simulink model "CHB_inverter_PEE_PROJECT"  (R2026a)
settings: Solver=VariableStepAuto  StopTime=0.04
libraries: nesl_utility x15, ee_lib x10, fl_lib x8, simulink x4
settings Model: Creator=THIRUPUGAZHL S D  LastModifiedBy=THIRUPUGAZHL S D

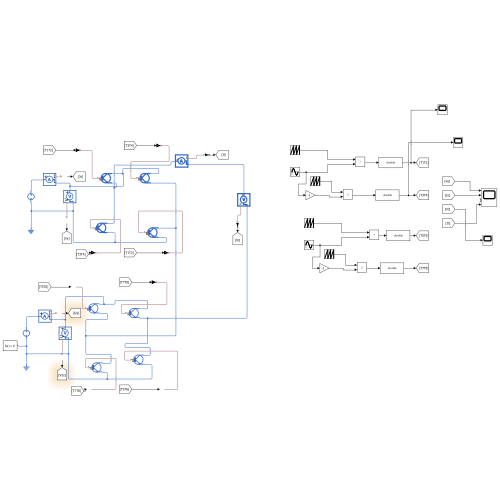
[thumbnail: Simulink's stored preview of the top-level diagram]
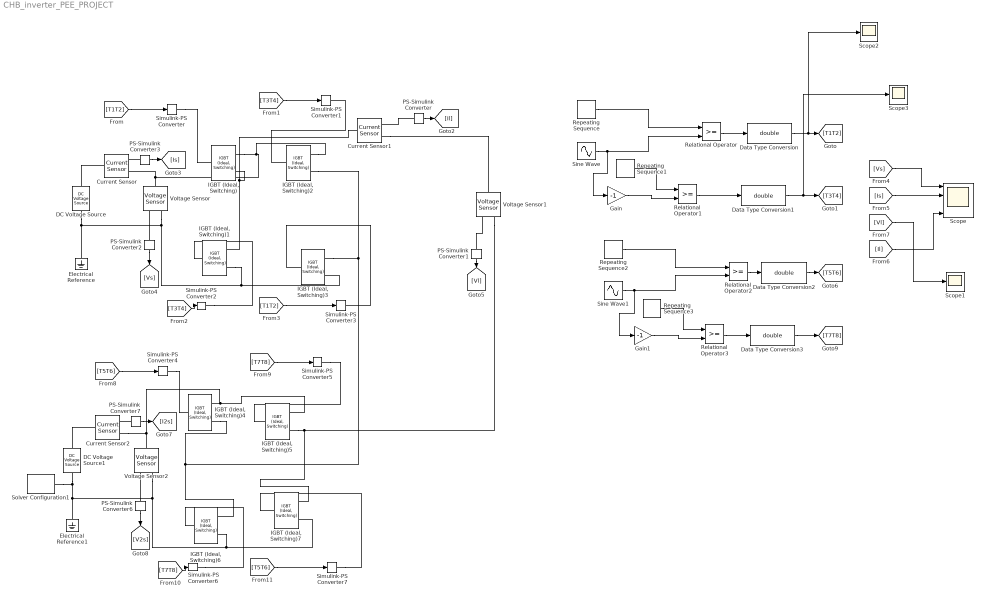
== system CHB_inverter_PEE_PROJECT ==
  Current Sensor : fl_lib/Electrical/Electrical Sensors/Current Sensor
  Current Sensor1 : fl_lib/Electrical/Electrical Sensors/Current Sensor
  Current Sensor2 : fl_lib/Electrical/Electrical Sensors/Current Sensor
  DC Voltage Source : ee_lib/Additional Components/SPICE Sources/DC Voltage Source  DC=50 V
  DC Voltage Source1 : ee_lib/Additional Components/SPICE Sources/DC Voltage Source  DC=50 V
  Data Type Conversion{,1..3} (4 alike) : DataTypeConversion  OutDataTypeStr=double  SaturateOnIntegerOverflow=off  RndMeth=Floor
  Electrical Reference : fl_lib/Electrical/Electrical Elements/Electrical Reference
  Electrical Reference1 : fl_lib/Electrical/Electrical Elements/Electrical Reference
  Gain : Gain  Gain=-1
  Gain1 : Gain  Gain=-1
  IGBT (Ideal, Switching){,1..7} (8 alike) : ee_lib/Semiconductors & Converters/IGBT (Ideal, Switching)  port_option=ee.enum.controlport.ps  Vf=0.8 V  Ron=0.001 Ohm  Goff=1e-5 1/Ohm  Vth=0.5 V  diode_param=ee.enum.semiconductors.protectionDiode.external  diode_Vf=0.8 V  diode_Ron=0.001 Ohm  diode_Goff=1e-5 1/Ohm  diode_C=50e-9 F  diode_iRM=-235 A  diode_iF=300 A  diode_idot=-50 A/us  diode_trr_param=ee.enum.converters.diodeReverseParam.trr_factor  diode_trr_factor=3  diode_trr=15 us  diode_Qrr=1500 s*uA  ice_specify=off  ice_priority=None  ice=0 A  ice_nominal_specify=off  ice_nominal_value=1  ice_nominal_unit=A  vce_specify=off  vce_priority=None  vce=0 V  vce_nominal_specify=off  vce_nominal_value=1  vce_nominal_unit=V  vge_specify=off  vge_priority=None  vge=0 V  vge_nominal_specify=off  vge_nominal_value=1  vge_nominal_unit=V  thermal_loss_option=ee.enum.converters.thermalLossOption.constantvalues  Von_data=[0, .1, .6, .8, 1, 1.3, 1.6, 2, 2.4; 0, .1, .7, 1, 1.2, 1.5, 1.9, 2.4, 2.8] V  Tj=[298.15, 398.15] K  Iout_data=[0, .1, 1, 5, 10, 20, 40, 70, 100] A  tabulateWithVce=false  Eon_data=[0, .0024, .024, .12, .2, .48, 1.04, 2.16, 3.24; 0, .003, .03, .15, .25, .6, 1.3, 2.7, 4.05] * 1e-3 J  Eoff_data=[0, .0007, .0066, .033, .066, .17, .33, .83, 1.5; 0, .001, .01, .05, .1, .25, .5, 1.2, 2.2] * 1e-3 J  Eon_data_3D=[zeros(2, 9, 3)] J  Eoff_data_3D=[zeros(2, 9, 3)] J  Tj_loss=[298.15, 398.15] K  Iout_data_loss=[0, .1, 1, 5, 10, 20, 40, 70, 100] A  Vce_loss=[0, 150, 300] V  Eon_scalar=22.86e-3 J  Eoff_scalar=17.14e-3 J  Voff=300 V  Iout_scalar=600 A  useCurrentFromPreviousCycle=false  useVoltageFromPreviousCycle=false  diodeModelType=ee.enum.converters.diodeModelType.pwl  diodeTableType=ee.enum.diode.tableType.IfMat  diode_ReverseIVType=ee.enum.diode.diodeReverseIV.constant  diode_IfMat=[.07, .12, .19, 1.75, 4.24, 7.32, 11.2; .16, .3, .72, 2.14, 4.02, 6.35, 9.12] A  diode_VfMat=[.9, 1.15, 1.25, 1.5, 1.75, 2.17, 2.6, 2.85; .58, .68, .75, 1.1, 1.38, 1.77, 2.27, 2.7] V  diode_TjVec=[25, 125] degC  diode_VfVec=[.5, .7, .9, 1.3, 1.7, 2.1, 2.5] V  diode_IfVec=[.1, .2, .5, 1, 2, 4, 7, 10] A  diode_IrMat=[1e-06, 2e-06, 5e-06, 1e-05, 2.5e-05, 5e-05, .0001; 2e-06, 5e-06, 1e-05, 4e-05, 8e-05, .0002, .0005] A  diode_VrMat=[10, 100, 200, 250, 300, 325, 350; 10, 70, 160, 220, 270, 300, 320] V  diode_VrVec=[10, 20, 40, 50, 70, 80, 100] V  diode_IrVec=[1e-06, 2e-06, 5e-06, 1e-05, 2e-05, 5e-05, .0001] A  diode_Vr=-600 V  diode_Ls=150 nH  diode_Erec=0.03 J  diode_rec_loss_model=ee.enum.diode.reverseRecoveryModelTabulateUpTo3D.fixed  diode_ErecVal=0 J  diode_scaleWithIandV=true  diode_ErecMat=zeros(2, 3) J  diodeErecMat3D=zeros(2, 3, 2) J  diode_TjrecVec=[298.15, 398.15] K  diode_IfrecVec=[.1, 1, 10] A  diodeVrecVec=[0, 100] V  diode_IrecVal=10 A  diode_VrecVal=10 V  diode_tFilter=1 / 1000 / 100 s  separateThermalPortForDiode=false  thermal_network_parameterization=ee.enum.thermalNetworkTopology.external  Rth=[.08, .5] K/W  Rth_Cauer=[.08, .1, .5] K/W  Rth_Foster=[.08, .14, .22, .16] K/W  thermal_mass_parameterization=ee.enum.thermalNetwork.timeconstant  thermal_mass=[.01, .5] J/K  thermal_mass_Cauer=[.01, .1, .5] J/K  thermal_mass_Foster=[.001, .005, .05, .5] J/K  thermal_time_constant=[.001, .2] s  thermal_time_constant_Cauer=[.001, .1, .2] s  thermal_time_constant_Foster=[7e-05, .0007, .01, .08] s  thermal_mass_initial_temperatures=[25, 25] degC  thermal_mass_initial_temperatures_Cauer=[25, 25, 25] degC  junction_thermal_mass=0.01 J/K  Tvec_initial_Foster=[25, 25, 25, 25] degC  RthDiode=[.03, .2] K/W  RthCauerDiode=[.03, .1, .2] K/W  RthFosterDiode=[.03, .2] K/W  thermalMassDiode=[3, 25] J/K  thermalMassCauerDiode=[3, 10, 25] J/K  thermalMassFosterDiode=[33, 50] J/K  thermalTauDiode=[.1, 5] s  thermalTauCauerDiode=[.1, 1, 5] s  thermalTauFosterDiode=[1, 10] s  thermalMassInitTempDiode=[25, 25] degC  thermalMassInitTempCauerDiode=[25, 25, 25] degC  junctionthermalMassDiode=0.1 J/K  TVecInitialFosterDiode=[25, 25, 25, 25] degC  no_thermal_network=ee.enum.enable.no  IGBT_junction_temperature_specify=off  IGBT_junction_temperature_priority=None  IGBT_junction_temperature=25 degC  IGBT_junction_temperature_nominal_specify=off  IGBT_junction_temperature_nominal_value=1  IGBT_junction_temperature_nominal_unit=degC  diode_junction_temperature_specify=off  diode_junction_temperature_priority=None  diode_junction_temperature=25 degC  diode_junction_temperature_nominal_specify=off  diode_junction_temperature_nominal_value=1  diode_junction_temperature_nominal_unit=degC  Qj_specify=off  Qj_priority=None  Qj=0 W  Qj_nominal_specify=off  Qj_nominal_value=1  Qj_nominal_unit=W  accumulatedSwitchingLosses_specify=off  accumulatedSwitchingLosses_priority=None  accumulatedSwitchingLosses=0 J
  PS-Simulink Converter{,1..3,6..7} (6 alike) : nesl_utility/PS-Simulink Converter  PhysicalDomain=network_engine_domain  SubClassName=ps_output  LeftPortType=input  RightPortType=output  PseudoPeriodic=off  Frequencies=[]  VectorFormat=inherit  Unit=inherit  AffineConversion=off
  Relational Operator{,1..3} (4 alike) : RelationalOperator  OutDataTypeStr=boolean  RndMeth=Simplest  InputSameDT=off
  Repeating Sequence : simulink/Sources/Repeating Sequence  rep_seq_t=[0 1]  rep_seq_y=[0 1]
  Repeating Sequence1 : simulink/Sources/Repeating Sequence  rep_seq_t=[0 1]  rep_seq_y=[0 1]
  Repeating Sequence2 : simulink/Sources/Repeating Sequence  rep_seq_t=[0 1]  rep_seq_y=[1 2]
  Repeating Sequence3 : simulink/Sources/Repeating Sequence  rep_seq_t=[0 1]  rep_seq_y=[1 2]
  Scope : Scope  NumInputPorts=4
      settings: ActiveDisplayYMinimum=40  ActiveDisplayYMaximum=60
  Scope1 : Scope
      settings: ActiveDisplayYMinimum=-60.499998790000006  ActiveDisplayYMaximum=60.499998790000006
  Scope2 : Scope
      settings: ActiveDisplayYMinimum=-1  ActiveDisplayYMaximum=1  DataLoggingVariableName=ScopeData2
  Scope3 : Scope
      settings: ActiveDisplayYMinimum=-0.12499999999999997  ActiveDisplayYMaximum=1.125  DataLoggingVariableName=ScopeData3
  Simulink-PS Converter{,1..7} (8 alike) : nesl_utility/Simulink-PS Converter  PhysicalDomain=network_engine_domain  SubClassName=ps_input  LeftPortType=input  RightPortType=output  PseudoPeriodic=off  Frequencies=[]  NoiseDistribution=none  NoiseParameters=[]  Unit=1  AffineConversion=off  FilteringAndDerivatives=provide  SimscapeFilterOrder=1  InputFilterTimeConstant=0.001  UdotUserProvided=0
  Sine Wave : Sin  Amplitude=2  Frequency=314  SampleTime=0
  Sine Wave1 : Sin  Amplitude=2  Frequency=314  SampleTime=0
  Solver Configuration1 : nesl_utility/Solver Configuration  PhysicalDomain=network_engine_domain  SubClassName=solver  LeftPortType=input  RightPortType=generic  Tones=[]  Harmonics=[]  SimulateNoise=off  Profile=off  UseLocalSampling=off  EnableSwitchedLinearOptims=on  FrequencyDomain=off  UseCCode=off  RelTol=0.001  AbsTol=0.001  MinStep=1e-09  ToWorkspace=off  RevertToSquareIcSolve=off  NumHomotopyIterations=100  PhasorMode=off  PhasorModeNumHarmonics=1  ConsistencySolver=NEWTON_XTOL_AFTER_FTOL  CanonicalOrdering=CANONICAL  OptimizeIntermediates=OPTIMIZED  IndexReductionMethod=DerivativeReplacement  DoDC=off  ResidualTolerance=1e-09  ConsistencyTolSource=GLOBAL  ConsistencyAbsTol=0.001  ConsistencyRelTol=0.001  ConsistencyTolFactor=0.001  UseLocalSolver=off  LocalSolverChoice=NE_BACKWARD_EULER_ADVANCER  ResolveIndetEquations=on  FunctionEvalNumThread=1  LocalSolverSampleTime=0.001  DoFixedCost=off  MaxNonlinIter=3  MaxModeIter=2  ComputeImpulses=off  ImpulseIterations=2  LinearAlgebra=auto  LinearAlgebraNumThread=0  EquationFormulation=NE_TIME_EF  DelaysMemoryBudget=1024  AutomaticFiltering=on  FilteringTimeConstant=0.001  PartitionStorageMethod=AS_NEEDED  PartitionMemoryBudget=1024  PartitionMethod=ROBUST  MultibodyUseLocalSolver=off  MultibodyLocalSolverChoice=ODE1  MultibodyLocalSolverSampleTime=0.001
  Voltage Sensor : fl_lib/Electrical/Electrical Sensors/Voltage Sensor
  Voltage Sensor1 : fl_lib/Electrical/Electrical Sensors/Voltage Sensor
  Voltage Sensor2 : fl_lib/Electrical/Electrical Sensors/Voltage Sensor
  wires:
  [T1T2] -> Simulink-PS Converter/1
  PS-Simulink Converter/1 -> [Il]
  PS-Simulink Converter2/1 -> [Vs]
  PS-Simulink Converter3/1 -> [Is]
  [T3T4] -> Simulink-PS Converter1/1
  PS-Simulink Converter1/1 -> [Vl]
  [Vs] -> Scope/1
  [T1T2] -> Simulink-PS Converter3/1
  [Il] -> Scope/4
  [T3T4] -> Simulink-PS Converter2/1
  [Is] -> Scope/2
  [T7T8] -> Simulink-PS Converter5/1
  PS-Simulink Converter6/1 -> [V2s]
  [T5T6] -> Simulink-PS Converter7/1
  PS-Simulink Converter7/1 -> [I2s]
  [T7T8] -> Simulink-PS Converter6/1
  [T5T6] -> Simulink-PS Converter4/1
  Repeating Sequence/1 -> Relational Operator/1
  Sine Wave/1 -> Gain/1, Relational Operator/2
  Repeating Sequence1/1 -> Relational Operator1/1
  Gain/1 -> Relational Operator1/2
  Gain1/1 -> Relational Operator3/2
  Repeating Sequence3/1 -> Relational Operator3/1
  Repeating Sequence2/1 -> Relational Operator2/1
  Sine Wave1/1 -> Gain1/1, Relational Operator2/2
  Relational Operator/1 -> Data Type Conversion/1
  Relational Operator1/1 -> Data Type Conversion1/1
  Relational Operator3/1 -> Data Type Conversion3/1
  Relational Operator2/1 -> Data Type Conversion2/1
  Data Type Conversion/1 -> Scope2/1, [T1T2]
  Data Type Conversion1/1 -> Scope3/1, [T3T4]
  Data Type Conversion2/1 -> [T5T6]
  Data Type Conversion3/1 -> [T7T8]
  [Vl] -> Scope1/1
  connections:
  Current Sensor1/RConn2 -- Voltage Sensor1/LConn1
  Simulink-PS Converter2/RConn1 -- "IGBT (Ideal, Switching)1"/LConn1
  PS-Simulink Converter1/LConn1 -- Voltage Sensor1/RConn1
  PS-Simulink Converter2/LConn1 -- Voltage Sensor/RConn1
  Simulink-PS Converter/RConn1 -- "IGBT (Ideal, Switching)"/LConn1
  "IGBT (Ideal, Switching)2"/LConn1 -- Simulink-PS Converter1/RConn1
  PS-Simulink Converter/LConn1 -- Current Sensor1/RConn1
  PS-Simulink Converter3/LConn1 -- Current Sensor/RConn1
  DC Voltage Source/LConn1 -- Current Sensor/LConn1
  "IGBT (Ideal, Switching)3"/LConn1 -- Simulink-PS Converter3/RConn1
  "IGBT (Ideal, Switching)4"/RConn1 -- Voltage Sensor2/LConn1 -- Current Sensor2/RConn2 -- "IGBT (Ideal, Switching)5"/RConn1
  PS-Simulink Converter6/LConn1 -- Voltage Sensor2/RConn1
  Simulink-PS Converter5/RConn1 -- "IGBT (Ideal, Switching)5"/LConn1
  PS-Simulink Converter7/LConn1 -- Current Sensor2/RConn1
  Simulink-PS Converter4/RConn1 -- "IGBT (Ideal, Switching)4"/LConn1
  Simulink-PS Converter7/RConn1 -- "IGBT (Ideal, Switching)7"/LConn1
  DC Voltage Source1/LConn1 -- Current Sensor2/LConn1
  Simulink-PS Converter6/RConn1 -- "IGBT (Ideal, Switching)6"/LConn1
  "IGBT (Ideal, Switching)6"/RConn2 -- Solver Configuration1/RConn1 -- DC Voltage Source1/RConn1 -- Electrical Reference1/LConn1 -- Voltage Sensor2/RConn2 -- "IGBT (Ideal, Switching)7"/RConn2
  "IGBT (Ideal, Switching)"/RConn2 -- "IGBT (Ideal, Switching)1"/RConn1 -- Current Sensor1/LConn1
  Voltage Sensor/LConn1 -- "IGBT (Ideal, Switching)2"/RConn1 -- "IGBT (Ideal, Switching)"/RConn1 -- Current Sensor/RConn2
  "IGBT (Ideal, Switching)1"/RConn2 -- Electrical Reference/LConn1 -- DC Voltage Source/RConn1 -- Voltage Sensor/RConn2 -- "IGBT (Ideal, Switching)3"/RConn2
  "IGBT (Ideal, Switching)4"/RConn2 -- "IGBT (Ideal, Switching)2"/RConn2 -- "IGBT (Ideal, Switching)3"/RConn1 -- "IGBT (Ideal, Switching)6"/RConn1
  "IGBT (Ideal, Switching)5"/RConn2 -- Voltage Sensor1/RConn2 -- "IGBT (Ideal, Switching)7"/RConn1
